simulink model "hdlcoder_dti_eml"  (R2026a)
settings: Solver=FixedStepDiscrete  StopTime=1000  FixedStep=1
InitFcn:
  | if ~exist('init_val'), init_val =  1; end;
  | if ~exist('gain_val'), gain_val =  1; end;
  | if ~exist('upper_limit'), upper_limit =  2; end;
  | if ~exist('lower_limit'), lower_limit =  0; end;
StopFcn:
  | disp('Successfully ran simulation')
  | disp('Results matched for the following settings')
  | disp('%%%%%%%%% Parameter Values %%%%%%%%%');
  | init_val
  | gain_val
  | upper_limit
  | lower_limit
undefined symbols (not defined in the file or in its folder): DiscIntNeverNeededParam, gain_val, init_val, lower_limit, upper_limit
libraries: dspsrcs4 x1
settings Model: Creator=The MathWorks, Inc.  LastModifiedBy=The MathWorks, Inc.
settings OptimizationCC: ConditionallyExecuteInputs=off  InitFltsAndDblsToZero=on
settings DebuggingCC: AlgebraicLoopMsg=error  SaveWithParameterizedLinksMsg=none  MultiTaskDSMMsg=warning  MultiTaskCondExecSysMsg=none  SingleTaskRateTransMsg=error
settings HardwareCC: ProdHWDeviceType=Specified
settings GRTTargetCC: TargetFcnLib=ansi_tfl_tmw.mat  CombineOutputUpdateFcns=off  GRTInterface=on

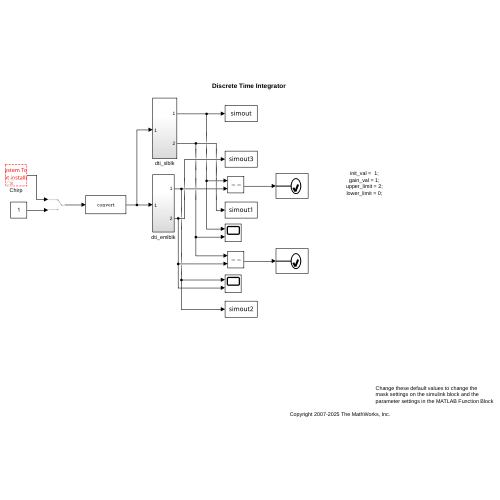
[thumbnail: Simulink's stored preview of the top-level diagram]
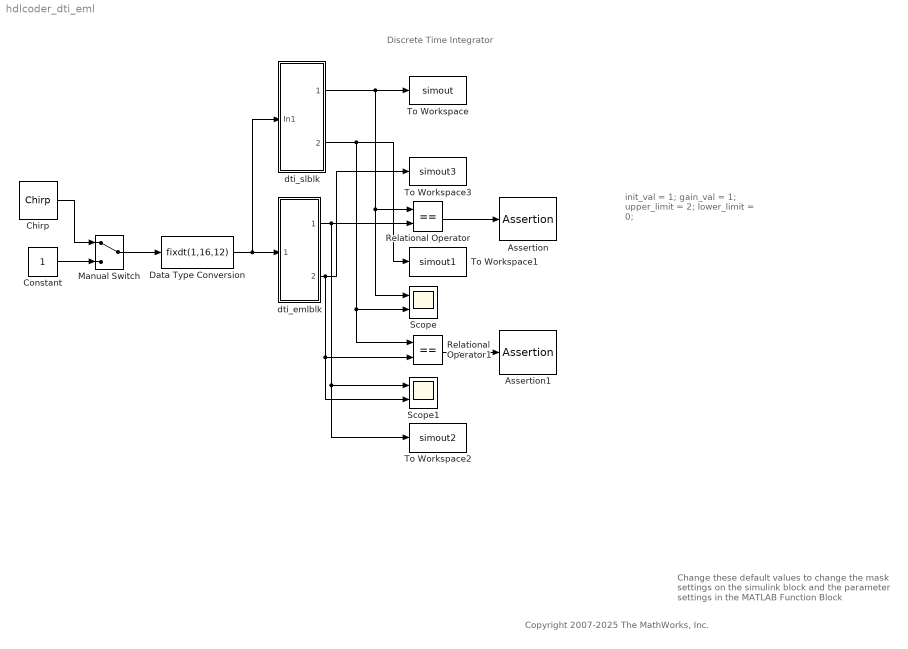
== system hdlcoder_dti_eml ==
  note: init_val =  1;
      | gain_val = 1;
      | upper_limit = 2;
      | lower_limit = 0;
  note: Change these default values to change the
      | mask settings on the simulink block and the
      | parameter settings in the MATLAB Function Block
  note: Discrete Time Integrator
  note: Copyright 2007-2025 The MathWorks, Inc.
  Assertion : Assertion
  Assertion1 : Assertion
  Chirp : dspsrcs4/Chirp  sweep=Linear  mode=Unidirectional  f0=0.1  f1=1  t1=100  Tsweep=100  phase=0  Ts=1  spf=1  datatype=double  OutputFrames=off
  Constant : Constant  SampleTime=1
  Data Type Conversion : DataTypeConversion  OutDataTypeStr=fixdt(1,16,12)  SaturateOnIntegerOverflow=off  RndMeth=Floor
  Manual Switch : ManualSwitch
  Relational Operator : RelationalOperator  Operator===  OutDataTypeStr=boolean  InputSameDT=off
  Relational Operator1 : RelationalOperator  Operator===  OutDataTypeStr=boolean  InputSameDT=off
  Scope : Scope  NumInputPorts=2
      settings: ActiveDisplayYMinimum=0  ActiveDisplayYMaximum=2
  Scope1 : Scope  NumInputPorts=2
      settings: ActiveDisplayYMinimum=0  ActiveDisplayYMaximum=2
  To Workspace : ToWorkspace  VariableName=simout  SampleTime=-1
  To Workspace1 : ToWorkspace  VariableName=simout1  SampleTime=-1
  To Workspace2 : ToWorkspace  VariableName=simout2  SampleTime=-1
  To Workspace3 : ToWorkspace  VariableName=simout3  SampleTime=-1
  dti_emlblk : Subsystem
  dti_slblk : Subsystem
  wires:
  Chirp/1 -> Manual Switch/1
  Constant/1 -> Manual Switch/2
  Relational Operator1/1 -> Assertion1/1
  Relational Operator/1 -> Assertion/1
  Manual Switch/1 -> Data Type Conversion/1
  Data Type Conversion/1 -> dti_emlblk/1(In1), dti_slblk/1(In1)
  dti_slblk/2(Out2) -> Scope/2, Relational Operator1/1, To Workspace1/1
  dti_slblk/1(Out1) -> Relational Operator/1, Scope/1, To Workspace/1
  dti_emlblk/2(Out2) -> Relational Operator1/2, Scope1/2, To Workspace3/1
  dti_emlblk/1(Out1) -> To Workspace2/1, Scope1/1, Relational Operator/2

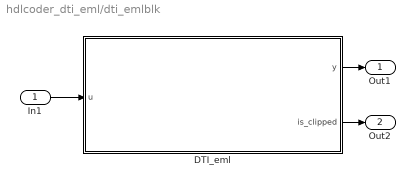
== system hdlcoder_dti_eml/dti_emlblk ==
  In1 : Inport
  DTI_eml : MATLAB Function  TreatAsAtomicUnit=on
  Out1 : Outport
  Out2 : Outport  Port=2
  wires:
  In1/1 -> DTI_eml/1(u)
  DTI_eml/1(y) -> Out1/1
  DTI_eml/2(is_clipped) -> Out2/1

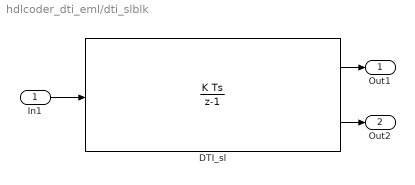
== system hdlcoder_dti_eml/dti_slblk ==
  In1 : Inport
  DTI_sl : DiscreteIntegrator  gainval=gain_val  InitialCondition=init_val  OutDataTypeStr=fixdt(1,16,12)  LimitOutput=on  UpperSaturationLimit=upper_limit  LowerSaturationLimit=lower_limit  ShowSaturationPort=on  ICPrevOutput=DiscIntNeverNeededParam  ICPrevScaledInput=DiscIntNeverNeededParam
  Out1 : Outport
  Out2 : Outport  Port=2
  wires:
  In1/1 -> DTI_sl/1
  DTI_sl/1 -> Out1/1
  DTI_sl/2 -> Out2/1

== matlab function hdlcoder_dti_eml/dti_emlblk/DTI_eml ==
  settings: updateMethod=DISCRETE  sampleTime=1
  settings: fimath=|
      | fimath(...
      | 'RoundMode', 'floor',...
      | 'OverflowMode', 'wrap',...
      | 'ProductMode', 'FullPrecision', 'ProductWordLength', 32,...
      | 'SumMode', 'FullPrecision', 'SumWordLength', 32,...
      | 'CastBeforeSum', true)
  data: u input; y output; init_val parameter; gain_val parameter; upper_limit parameter; lower_limit parameter; is_clipped output
function [y, is_clipped] = fcn(u, init_val, gain_val, upper_limit, lower_limit)
% Discrete Time Integrator in MATLAB Function block

%
% Forward Euler method, also known as Forward Rectangular, 
% or left-hand approximation.  The resulting expression for the 
% output of the block at step n is
%
% y(n) = y(n-1) + K * u(n-1)
%


%%%%%%%%%%%
% Setup
%%%%%%%%%%%

% numeric type to clip the accumulator value after each addition
nt = numerictype(u);
fm = fimath(u);

% variable to hold state between consecutive calls to this block
persistent u_state;
if isempty(u_state)
    u_state = fi(init_val, nt, fm);
end

% numeric type to represent -1,1,0 (sfix2)
nt2 = numerictype(1, 2, 0);

% clip flag status
positive_sat_occurred = fi(1, nt2, fm);
negative_sat_occurred = fi(-1, nt2, fm);
no_sat_occurred = fi(0, nt2, fm);

% cast matlab parameters to proper types
gv = fi(gain_val, nt, fm);
ul = fi(upper_limit, nt, fm);
ll = fi(lower_limit, nt, fm);


%%%%%%%%%%%%%%%%%
% Compute Output
%%%%%%%%%%%%%%%%%

if (u_state >= ul)
    t = ul;
    is_clipped = positive_sat_occurred;
elseif (u_state <= ll)
	t = ll;
    is_clipped = negative_sat_occurred;
else    
    t = u_state;
    is_clipped = no_sat_occurred;
end

y = t;


%%%%%%%%%%%%%%%%%
% Update State
%%%%%%%%%%%%%%%%%

tprod = fi(gv * u, nt, fm);
u_state = fi(t + tprod, nt, fm);
